simulink model "PEproject_PredictiveMaintenance"  (R2025a)
settings: Solver=VariableStepAuto  StartTime=0.0  StopTime=10  RelTol=1e-3
InitFcn:
  | pm_setup
values from neighbouring files (symbols this model uses):
  N = size(S,1);  fprintf('    [pm_generate_data.m]
  PM = S.PM;  PM.trained = true    [pm_setup.m]    (also in pm_train_model.m = PM0; pm_trained.mat = )
libraries: spsDCVoltageSourceLib x2, spsDiodeLib x2, spsDCMachineLib x1, spsIGBTLib x1, slpidlib x1, spsPWMGeneratorDCDCLib x1, spsSeriesRLCBranchLib x1, simulink x1, spspowerguiLib x1
settings DebuggingCC: UnconnectedInputMsg=warning  UnconnectedOutputMsg=warning  UnconnectedLineMsg=warning
settings ModelReferenceCC: EnableRefExpFcnMdlSchedulingChecks=on
settings RTWCC: GPUComputeCapability=3.5  DLArmComputeVersion=19.05

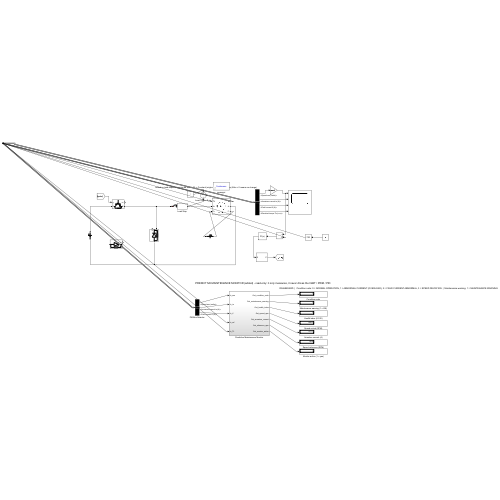
[thumbnail: Simulink's stored preview of the top-level diagram]
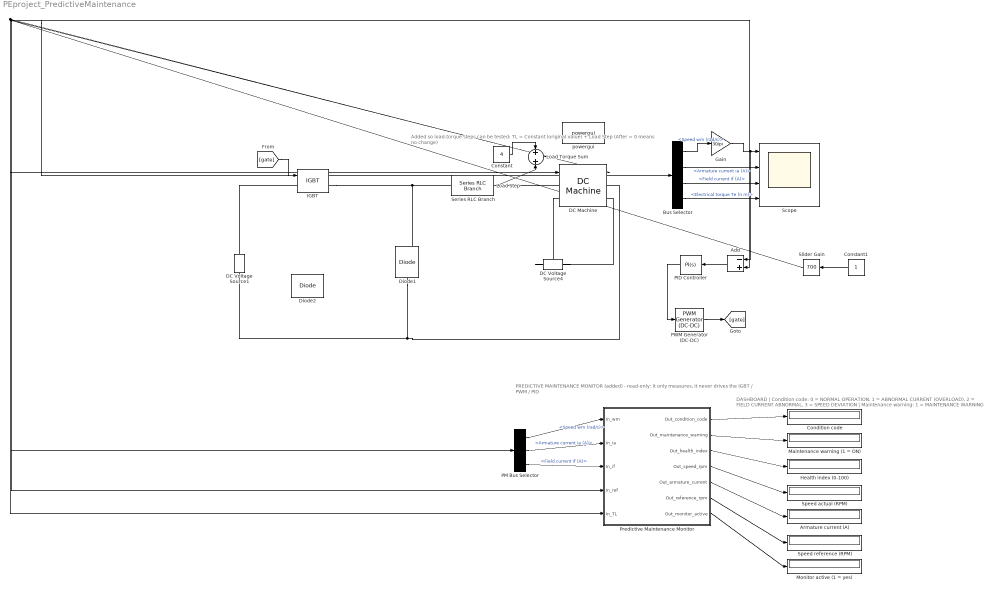
== system PEproject_PredictiveMaintenance ==
  note: PREDICTIVE MAINTENANCE MONITOR (added) - read-only: it only measures, it never drives the IGBT / PWM / PID
  note: DASHBOARD | Condition code: 0 = NORMAL OPERATION, 1 = ABNORMAL CURRENT (OVERLOAD), 2 = FIELD CURRENT ABNORMAL, 3 = SPEED DEVIATION | Maintenance warning: 1 = MAINTENANCE WARNING
  note: Added so load-torque steps can be tested: TL = Constant (original value) + Load Step (After = 0 means no change)
  Add : Sum  Inputs=-+
  Armature current (A) : Display
  Bus Selector : BusSelector  OutputSignals=Speed wm (rad/s),Armature current ia (A),Field current if (A),Electrical torque Te (n m)
  Condition code : Display
  Constant : Constant  Value=4
  Constant1 : Constant
  DC Machine : spsDCMachineLib/DC Machine  PresetModel=01: 5HP 240V 1750RPM Field:300V  MechanicalLoad=Torque TL  FieldType=Wound  ShowDetailedParameters=on  MeasurementBus=off  RLa=[2.581 0.028]  RLf=[281.2 156]  Laf=0.9483  MachineConstant=Torque constant (N.m/A)  Ke=1.8  Kt=1.8  J=0.02215  Bm=0.002953  Tf=0.5161  w0=1  Ifinit=1.06685633001422  TsPowergui=0  TsBlock=-1
  DC Voltage Source1 : spsDCVoltageSourceLib/DC Voltage Source  Amplitude=240  Measurements=None
  DC Voltage Source4 : spsDCVoltageSourceLib/DC Voltage Source  Amplitude=300  Measurements=None
  Diode1 : spsDiodeLib/Diode  Ron=0.001  Lon=0  Vf=0.8  IC=0  UseSnubber=0  Rs=500  Cs=250e-9  Measurements=on
  Diode2 : spsDiodeLib/Diode  Ron=0.001  Lon=0  Vf=0.8  IC=0  UseSnubber=0  Rs=500  Cs=250e-9  Measurements=on
  Gain : Gain  Gain=30/pi
  Health index (0-100) : Display
  IGBT : spsIGBTLib/IGBT  Ron=0.001  Lon=0  Vf=0  Tf=1e-6  Tt=2e-6  IC=0  Rs=1e5  Cs=inf  Measurements=on
  Load Step : Step  Time=5  After=0  SampleTime=0
  Load Torque Sum : Sum
  Maintenance warning (1 = ON) : Display
  Monitor active (1 = yes) : Display
  PID Controller : slpidlib/PID Controller  Controller=PI  Form=Parallel  TimeDomain=Continuous-time  UseExternalTs=off  SampleTime=-1  IntegratorMethod=Forward Euler  FilterMethod=Forward Euler  ControllerParametersSource=internal  P=2  I=12  UseKiTs=off  D=0  UseExternalDerivativeSource=off  N=100  UseFilter=on  TunerSelectOption=Transfer Function Based (PID Tuner App)  InitialConditionSource=internal  InitialConditionForIntegrator=0  InitialConditionForFilter=0  DifferentiatorICPrevScaledInput=0  ExternalReset=none  TrackingMode=off  Kt=1  LimitOutput=off  SatLimitsSource=internal  UpperSaturationLimit=inf  LowerSaturationLimit=-inf  LinearizeAsGain=on  AntiWindupMode=none  Kb=1  LimitIntegrator=off  UpperIntegratorSaturationLimit=inf  LowerIntegratorSaturationLimit=-inf  POutMin=[]  POutMax=[]  IOutMin=[]  IOutMax=[]  DOutMin=[]  DOutMax=[]  NOutMin=[]  NOutMax=[]  SumOutMin=[]  SumOutMax=[]  SaturationOutMin=[]  SaturationOutMax=[]  PParamMin=[]  PParamMax=[]  IParamMin=[]  IParamMax=[]  DParamMin=[]  DParamMax=[]  NParamMin=[]  NParamMax=[]  KbParamMin=[]  KbParamMax=[]  KtParamMin=[]  KtParamMax=[]  KbOutMin=[]  KbOutMax=[]  KtOutMin=[]  KtOutMax=[]  IntegratorOutMin=[]  IntegratorOutMax=[]  FilterOutMin=[]  FilterOutMax=[]  SumI1OutMin=[]  SumI1OutMax=[]  SumI2OutMin=[]  SumI2OutMax=[]  SumI3OutMin=[]  SumI3OutMax=[]  SumI4OutMin=[]  SumI4OutMax=[]  SumDOutMin=[]  SumDOutMax=[]  DifferentiatorOutMin=[]  DifferentiatorOutMax=[]  FilterDiffOutCoefMin=[]  FilterDiffOutCoefMax=[]  ReciprocalOutMin=[]  ReciprocalOutMax=[]  SumDenOutMin=[]  SumDenOutMax=[]  SumNumOutMin=[]  SumNumOutMax=[]  DivideOutMin=[]  DivideOutMax=[]  UdiffTsProdOutMin=[]  UdiffTsProdOutMax=[]  NTsProdOutMin=[]  NTsProdOutMax=[]  UintegralTsProdOutMin=[]  UintegralTsProdOutMax=[]  UngainTsProdOutMin=[]  UngainTsProdOutMax=[]  ClampingZeroOutDataTypeStr=Inherit: Inherit via back propagation  ClampingZeroOutMin=[]  ClampingZeroOutMax=[]  FilterDenConstantOutDataTypeStr=Inherit: Inherit via back propagation  FilterDenConstantOutMin=[]  FilterDenConstantOutMax=[]  PCopyOutDataTypeStr=Inherit: Inherit via back propagation  PCopyOutMin=[]  PCopyOutMax=[]  NCopyOutDataTypeStr=Inherit: Inherit via back propagation  NCopyOutMin=[]  NCopyOutMax=[]  IntegratorContinuousStateAttributes=''  IntegratorStateMustResolveToSignalObject=off  IntegratorRTWStateStorageClass=Auto  FilterContinuousStateAttributes=''  FilterStateMustResolveToSignalObject=off  FilterRTWStateStorageClass=Auto  ParallelPVariant=InternalParameters  IdealPVariant=Disabled  IVariant=InternalParameters  DVariant=Disabled  IntegratorVariant=Continuous  SatVariant=Disabled  AWVariant=Passthrough  PCopyVariant=Disabled  TRVariant=Disabled  FdbkBlocksVariant=Forward  IdealPFdbkVariant=Disabled  SatFdbkVariant=Disabled  DerivativeFilterVariant=Disabled  NVariant=Disabled  NCopyVariant=Disabled_SignalSpec  FilterICVariant=Disabled  IntegratorICVariant=InternalICs  ExternalResetVariant=Disabled  TRSumVariant=Passthrough  SumFdbkVariant=Disabled  SumVariant=Sum_PI  TsampFilterVariant=InternalTs  TsampNgainVariant=Passthrough  TsampIntegralVariant=Disabled_SignalSpec  ExternalSaturationOutDataTypeStr=Inherit: Same as second input  DerivativeSourceVariant=Disabled  PreIntVariant=InternalPreInt
  PM Bus Selector : BusSelector  OutputSignals=Speed wm (rad/s),Armature current ia (A),Field current if (A)
  PWM Generator (DC-DC) : spsPWMGeneratorDCDCLib/PWM Generator (DC-DC)  Fsw=2e3  Ts=0
  Predictive Maintenance Monitor : Subsystem
  Scope : Scope  NumInputPorts=4
      settings: ActiveDisplayYMinimum=-107.6996905255819  ActiveDisplayYMaximum=1057.7672674975424
  Series RLC Branch : spsSeriesRLCBranchLib/Series RLC Branch  LConnTagsString=__new0  RConnTagsString=__new0  BranchType=L  Resistance=1  Inductance=10e-3  SetiL0=off  InitialCurrent=0  Capacitance=1e-6  Setx0=off  InitialVoltage=0  Measurements=None
  Slider Gain : simulink/Math Operations/Slider Gain  gain=700  low=0  high=10000
  Speed actual (RPM) : Display
  Speed reference (RPM) : Display
  powergui : spspowerguiLib/powergui  Priority=1  SimulationMode=Continuous  SampleTime=50e-6  frequency=60  Iterations=50  frequencyindice=0  Pbase=100e6  ErrMax=1e-4  UnitsV=kV  UnitsW=MW  buscounter=0  FunctionMessages=off  echomessages=off  EnableUseOfTLC=off  CurrentSourceSwitches=off  DisableSnubberDevices=off  DisableRonSwitches=off  DisableVfSwitches=off  DisplayEquations=off  AutomaticDiscreteSolvers=off  SolverType=Tustin/Backward Euler (TBE)  Interpol=off  ExternalGateDelay=off  methode=off  Ts=100  x0status=blocks  SPID=on  SwTol=0  HookPort=off  NonlinearTolerance=1e-4  nMaxIteration=100  ContinueOnMaxIteration=off  RestoreLinks=warning  ResistiveCurrentMeasurement=off  Frange=[0:2:500]  Ylog=off  Xlog=on  ShowGrid=off  save=off  variable=ZData  structure=0  ZoomFFT=off  StartTime=0.0  cycles=1  DisplayStyle=1  fundamental=60  FreqAxis=off  MaxFrequency=1000  frequencyindicesteady=1  RmsSteady=1  display=off
  wires:
  DC Machine/1 -> Bus Selector/1, PM Bus Selector/1
  Bus Selector/2 -> Scope/2  "<Armature current ia (A)>"
  Bus Selector/1 -> Gain/1  "<Speed wm (rad/s)>"
  Bus Selector/3 -> Scope/3  "<Field current if (A)>"
  Bus Selector/4 -> Scope/4  "<Electrical torque Te (n m)>"
  Constant/1 -> Load Torque Sum/1
  Gain/1 -> Add/1, Scope/1
  Slider Gain/1 -> Add/2, Predictive Maintenance Monitor/4(In_ref)
  Constant1/1 -> Slider Gain/1
  Add/1 -> PID Controller/1
  [gate] -> IGBT/1
  PID Controller/1 -> PWM Generator (DC-DC)/1
  PWM Generator (DC-DC)/1 -> [gate]
  PM Bus Selector/1 -> Predictive Maintenance Monitor/1(In_wm)  "<Speed wm (rad/s)>"
  PM Bus Selector/2 -> Predictive Maintenance Monitor/2(In_ia)  "<Armature current ia (A)>"
  PM Bus Selector/3 -> Predictive Maintenance Monitor/3(In_if)  "<Field current if (A)>"
  Load Step/1 -> Load Torque Sum/2
  Load Torque Sum/1 -> DC Machine/1, Predictive Maintenance Monitor/5(In_TL)
  Predictive Maintenance Monitor/1(Out_condition_code) -> Condition code/1
  Predictive Maintenance Monitor/2(Out_maintenance_warning) -> Maintenance warning (1 = ON)/1
  Predictive Maintenance Monitor/3(Out_health_index) -> Health index (0-100)/1
  Predictive Maintenance Monitor/4(Out_speed_rpm) -> Speed actual (RPM)/1
  Predictive Maintenance Monitor/5(Out_armature_current) -> Armature current (A)/1
  Predictive Maintenance Monitor/6(Out_reference_rpm) -> Speed reference (RPM)/1
  Predictive Maintenance Monitor/7(Out_monitor_active) -> Monitor active (1 = yes)/1
  connections:
  Series RLC Branch/RConn1 -- DC Machine/LConn1
  IGBT/RConn1 -- Diode1/RConn1 -- Series RLC Branch/LConn1
  DC Voltage Source1/LConn1 -- DC Machine/RConn1 -- Diode1/LConn1
  DC Voltage Source4/RConn1 -- DC Machine/LConn2
  DC Voltage Source4/LConn1 -- DC Machine/RConn2
  DC Voltage Source1/RConn1 -- IGBT/LConn1

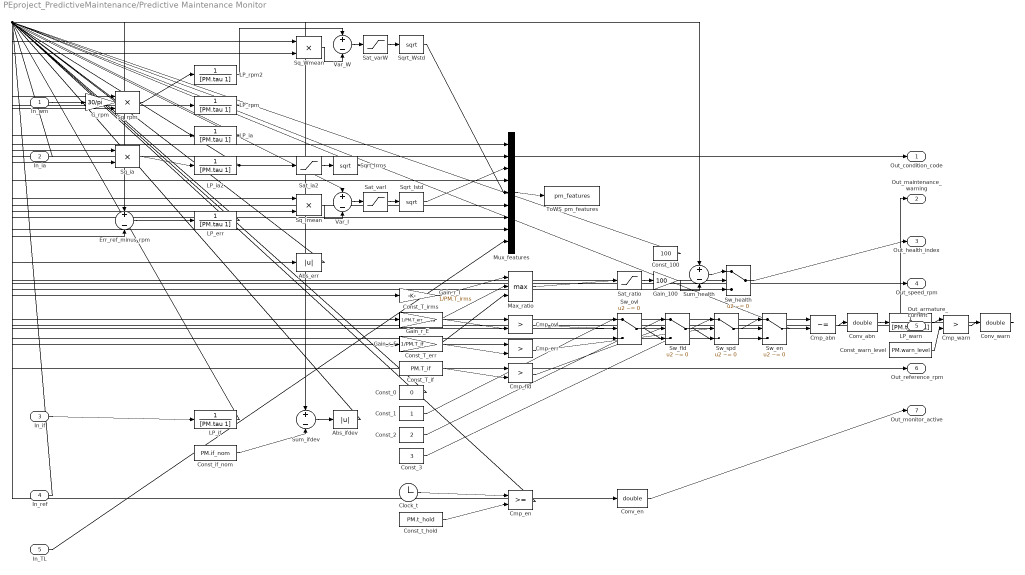
== system PEproject_PredictiveMaintenance/Predictive Maintenance Monitor ==
  In_wm : Inport
  In_ia : Inport  Port=2
  In_if : Inport  Port=3
  In_ref : Inport  Port=4
  In_TL : Inport  Port=5
  Abs_err : Abs
  Abs_ifdev : Abs
  Clock_t : Clock
  Cmp_abn : RelationalOperator  Operator=~=
  Cmp_en : RelationalOperator
  Cmp_err : RelationalOperator  Operator=>
  Cmp_fld : RelationalOperator  Operator=>
  Cmp_ovl : RelationalOperator  Operator=>
  Cmp_warn : RelationalOperator  Operator=>
  Const_0 : Constant  Value=0
  Const_1 : Constant
  Const_100 : Constant  Value=100
  Const_2 : Constant  Value=2
  Const_3 : Constant  Value=3
  Const_T_err : Constant  Value=PM.T_err
  Const_T_if : Constant  Value=PM.T_if
  Const_T_irms : Constant  Value=PM.T_irms
  Const_if_nom : Constant  Value=PM.if_nom
  Const_t_hold : Constant  Value=PM.t_hold
  Const_warn_level : Constant  Value=PM.warn_level
  Conv_abn : DataTypeConversion  OutDataTypeStr=double
  Conv_en : DataTypeConversion  OutDataTypeStr=double
  Conv_warn : DataTypeConversion  OutDataTypeStr=double
  Err_ref_minus_rpm : Sum  Inputs=+-
  G_rpm : Gain  Gain=30/pi
  Gain_100 : Gain  Gain=100
  Gain_r_E : Gain  Gain=1/PM.T_err
  Gain_r_F : Gain  Gain=1/PM.T_if
  Gain_r_I : Gain  Gain=1/PM.T_irms
  LP_err : TransferFcn  Denominator=[PM.tau 1]
  LP_ia : TransferFcn  Denominator=[PM.tau 1]
  LP_ia2 : TransferFcn  Denominator=[PM.tau 1]
  LP_if : TransferFcn  Denominator=[PM.tau 1]
  LP_rpm : TransferFcn  Denominator=[PM.tau 1]
  LP_rpm2 : TransferFcn  Denominator=[PM.tau 1]
  LP_warn : TransferFcn  Denominator=[PM.t_deb 1]
  Max_ratio : MinMax  Function=max  Inputs=3  InputSameDT=on  SaturateOnIntegerOverflow=on
  Mux_features : Mux  Inputs=9
  Sat_ia2 : Saturate  UpperLimit=inf  LowerLimit=0
  Sat_ratio : Saturate  UpperLimit=1  LowerLimit=0
  Sat_varI : Saturate  UpperLimit=inf  LowerLimit=0
  Sat_varW : Saturate  UpperLimit=inf  LowerLimit=0
  Sq_Imean : Product  InputSameDT=on  RndMeth=Zero  SaturateOnIntegerOverflow=on  OutDataTypeStr=Inherit: Same as first input
  Sq_Wmean : Product  InputSameDT=on  RndMeth=Zero  SaturateOnIntegerOverflow=on  OutDataTypeStr=Inherit: Same as first input
  Sq_ia : Product  InputSameDT=on  RndMeth=Zero  SaturateOnIntegerOverflow=on  OutDataTypeStr=Inherit: Same as first input
  Sq_rpm : Product  InputSameDT=on  RndMeth=Zero  SaturateOnIntegerOverflow=on  OutDataTypeStr=Inherit: Same as first input
  Sqrt_Irms : Sqrt
  Sqrt_Istd : Sqrt
  Sqrt_Wstd : Sqrt
  Sum_health : Sum  Inputs=+-
  Sum_ifdev : Sum  Inputs=+-
  Sw_en : Switch  Criteria=u2 ~= 0
  Sw_fld : Switch  Criteria=u2 ~= 0
  Sw_health : Switch  Criteria=u2 ~= 0
  Sw_ovl : Switch  Criteria=u2 ~= 0
  Sw_spd : Switch  Criteria=u2 ~= 0
  ToWS_pm_features : ToWorkspace  VariableName=pm_features  SaveFormat=Timeseries  SampleTime=-1
  Var_I : Sum  Inputs=+-
  Var_W : Sum  Inputs=+-
  Out_condition_code : Outport
  Out_maintenance_warning : Outport  Port=2
  Out_health_index : Outport  Port=3
  Out_speed_rpm : Outport  Port=4
  Out_armature_current : Outport  Port=5
  Out_reference_rpm : Outport  Port=6
  Out_monitor_active : Outport  Port=7
  wires:
  In_wm/1 -> G_rpm/1
  In_ia/1 -> Sq_ia/1, Sq_ia/2, LP_ia/1, Out_armature_current/1
  G_rpm/1 -> Sq_rpm/1, Sq_rpm/2, Err_ref_minus_rpm/2, LP_rpm/1, Out_speed_rpm/1
  In_ref/1 -> Err_ref_minus_rpm/1, Mux_features/8, Out_reference_rpm/1
  Sq_ia/1 -> LP_ia2/1
  Sq_rpm/1 -> LP_rpm2/1
  Err_ref_minus_rpm/1 -> LP_err/1
  In_if/1 -> LP_if/1
  LP_ia2/1 -> Var_I/1, Sat_ia2/1
  LP_ia/1 -> Sq_Imean/1, Sq_Imean/2, Mux_features/1
  Sq_Imean/1 -> Var_I/2
  LP_rpm/1 -> Sq_Wmean/1, Sq_Wmean/2, Mux_features/4
  LP_rpm2/1 -> Var_W/1
  Sq_Wmean/1 -> Var_W/2
  LP_err/1 -> Abs_err/1, Mux_features/6
  LP_if/1 -> Sum_ifdev/1, Mux_features/7
  Const_if_nom/1 -> Sum_ifdev/2
  Sum_ifdev/1 -> Abs_ifdev/1
  Sqrt_Irms/1 -> Mux_features/2, Cmp_ovl/1, Gain_r_I/1
  Sqrt_Istd/1 -> Mux_features/3
  Sqrt_Wstd/1 -> Mux_features/5
  In_TL/1 -> Mux_features/9
  Mux_features/1 -> ToWS_pm_features/1
  Const_T_irms/1 -> Cmp_ovl/2
  Abs_err/1 -> Cmp_err/1, Gain_r_E/1
  Const_T_err/1 -> Cmp_err/2
  Abs_ifdev/1 -> Cmp_fld/1, Gain_r_F/1
  Const_T_if/1 -> Cmp_fld/2
  Const_1/1 -> Sw_ovl/1
  Cmp_ovl/1 -> Sw_ovl/2
  Const_0/1 -> Sw_ovl/3, Sw_en/3, Cmp_abn/2
  Const_2/1 -> Sw_fld/1
  Cmp_fld/1 -> Sw_fld/2
  Sw_ovl/1 -> Sw_fld/3
  Const_3/1 -> Sw_spd/1
  Cmp_err/1 -> Sw_spd/2
  Sw_fld/1 -> Sw_spd/3
  Clock_t/1 -> Cmp_en/1
  Const_t_hold/1 -> Cmp_en/2
  Sw_spd/1 -> Sw_en/1
  Cmp_en/1 -> Sw_en/2, Sw_health/2, Conv_en/1
  Sw_en/1 -> Cmp_abn/1, Out_condition_code/1
  Cmp_abn/1 -> Conv_abn/1
  Conv_abn/1 -> LP_warn/1
  LP_warn/1 -> Cmp_warn/1
  Const_warn_level/1 -> Cmp_warn/2
  Cmp_warn/1 -> Conv_warn/1
  Gain_r_I/1 -> Max_ratio/1
  Gain_r_E/1 -> Max_ratio/2
  Gain_r_F/1 -> Max_ratio/3
  Const_100/1 -> Sum_health/1, Sw_health/3
  Gain_100/1 -> Sum_health/2
  Sum_health/1 -> Sw_health/1
  Conv_warn/1 -> Out_maintenance_warning/1
  Sw_health/1 -> Out_health_index/1
  Conv_en/1 -> Out_monitor_active/1
  Sat_ia2/1 -> Sqrt_Irms/1
  Max_ratio/1 -> Sat_ratio/1
  Sat_ratio/1 -> Gain_100/1
  Var_W/1 -> Sat_varW/1
  Sat_varW/1 -> Sqrt_Wstd/1
  Var_I/1 -> Sat_varI/1
  Sat_varI/1 -> Sqrt_Istd/1
